simulink model "My_gfm_datacenter_sil"  (R2018b)
settings: Solver=ode45  StartTime=0.0  StopTime=100  MaxStep=1e-4  RelTol=1e-3
PreLoadFcn:
  | modelDir = fileparts(get_param(bdroot,'FileName'));
  | 
  | load_system(fullfile(modelDir,'controls_element_lib.slx'));
  | load_system(fullfile(modelDir,'test_sequence_lib.slx'));
InitFcn:
  | close all;
  | clear all;
  | clc;
  | 
  | % frequency nominals
  | F_NOM = 60;
  | W_NOM = 2 * pi * F_NOM;
  | 
  | % base values relative to inverter
  | % --------------------------------
  | VLL_INV_NOM = 480;
  | P_INV_NOM = 1e6;
  | Q_INV_NOM = 0.5e6;
  | S_INV_NOM = sqrt(P_INV_NOM^2 + Q_INV_NOM^2);
  | 
  | I_INV_BASE = S_INV_NOM/(sqrt(3)*VLL_INV_NOM);
  | Z_INV_BASE = VLL_INV_NOM^2/S_INV_NOM;
  | L_INV_BASE = Z_INV_BASE / W_NOM;
  | C_INV_BASE = 1 / (Z_INV_BASE * W_NOM);
  | 
  | % nominal ratings for power system model
  | % --------------------------------------
  | INVERTER_COUNT = 100;
  | 
  | VLV_NOM = VLL_INV_NOM;
  | VMV_NOM = 35e3;
  | VHV_NOM = 230e3;
  | S_PLANT = INVERTER_COUNT * S_INV_NOM;
  | 
  | N_GSU = VHV_NOM/VMV_NOM;
  | N_MVT = VMV_NOM/VLV_NOM;
  | 
  | I_LV_BASE = S_PLANT/(sqrt(3)*VLV_NOM);
  | I_MV_BASE = S_PLANT/(sqrt(3)*VMV_NOM);
  | I_HV_BASE = S_PLANT/(sqrt(3)*VHV_NOM);
  | 
  | Z_LV_BASE = VLV_NOM^2/S_PLANT;
  | Z_MV_BASE = VMV_NOM^2/S_PLANT;
  | Z_HV_BASE = VHV_NOM^2/S_PLANT;
  | 
  | L_LV_BASE = Z_LV_BASE / W_NOM;
  | L_MV_BASE = Z_MV_BASE / W_NOM;
  | L_HV_BASE = Z_HV_BASE / W_NOM;
  | C_LV_BASE = 1 / (Z_LV_BASE * W_NOM);
  | C_MV_BASE = 1 / (Z_MV_BASE * W_NOM);
  | C_HV_BASE = 1 / (Z_HV_BASE * W_NOM);
undefined symbols (not defined in the file): C_BBU, C_MV_CELL, IDC_NOM, ILV_MAX, ILV_MIN, IMV_MAX, IMV_MIN, N_CELLS_PER_STRING, N_DCDC_XFMR, r_BBU, V_LVDC_NOM
libraries: test_sequence_lib x14, controls_element_lib x10, simulink x1
settings Model: SimulationMode=accelerator  Creator=HussamAlatrash  LastModifiedBy=ahhei
settings DataIOCC: ReturnWorkspaceOutputs=on
settings OptimizationCC: EfficientMapNaN2IntZero=off
settings DebuggingCC: UnconnectedInputMsg=none  UnconnectedOutputMsg=none  UnconnectedLineMsg=none
settings HardwareCC: TargetBitPerPointer=64  TargetBitPerSizeT=64  TargetBitPerPtrDiffT=64  TargetLongLongMode=on  TargetIntDivRoundTo=Zero  TargetEndianess=LittleEndian  TargetWordSize=64  TargetHWDeviceType=MATLAB Host  ProdEqTarget=off
settings ModelReferenceCC: EnableRefExpFcnMdlSchedulingChecks=off
settings CodeAppCC: MaxIdLength=128
settings GRTTargetCC: TargetLangStandard=C89/C90 (ANSI)  CombineOutputUpdateFcns=off  GRTInterface=on

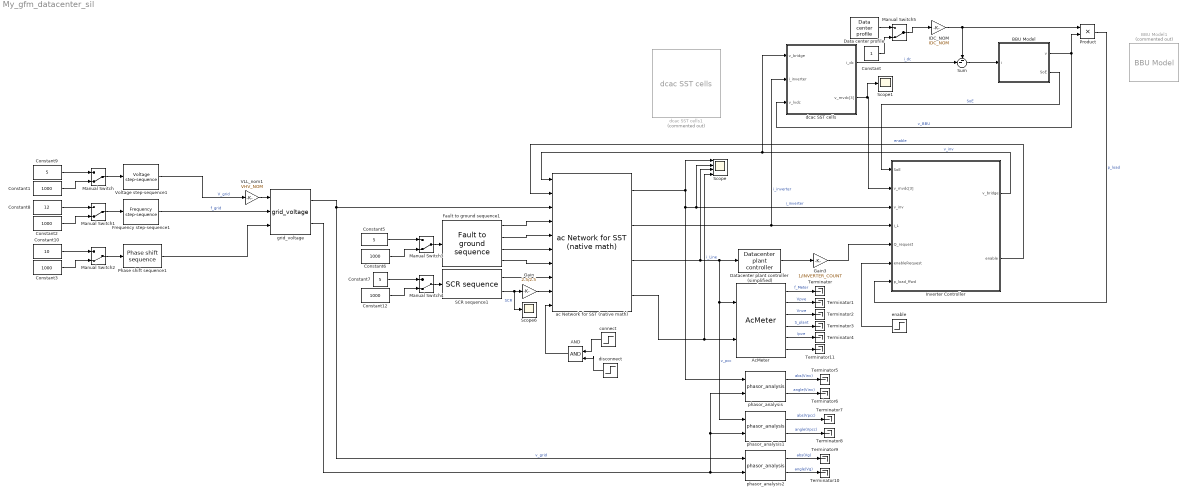
== system My_gfm_datacenter_sil ==
  AND : Logic  IconShape=distinctive  AllPortsSameDT=off  OutDataTypeStr=boolean
  AcMeter : test_sequence_lib/AcMeter  VllRated=VHV_NOM
  BBU Model : Subsystem  AncestorBlock=test_sequence_lib/BBU Model
  BBU Model1 : test_sequence_lib/BBU Model  Commented=on  SystemSampleTime=-1
  Constant : Constant
  Constant{1..3,6,12} (5 alike) : Constant  Value=1000
  Constant10 : Constant  Value=10
  Constant5 : Constant  Value=5
  Constant7 : Constant  Value=5
  Constant8 : Constant  Value=12
  Constant9 : Constant  Value=5
  Data center profile : test_sequence_lib/Data center profile  SystemSampleTime=-1
  Datacenter plant controller (simplified) : controls_element_lib/Datacenter plant controller  SystemSampleTime=-1
  Fault to ground sequence1 : test_sequence_lib/Fault to ground sequence  SystemSampleTime=-1
  Frequency step-sequence1 : test_sequence_lib/Frequency step-sequence  SystemSampleTime=-1
  Gain : Gain  Gain=2.5/2.5
  Gain3 : Gain  Gain=1/INVERTER_COUNT
  IDC_NOM : Gain  Gain=IDC_NOM
  Inverter Controller : Subsystem
  Manual Switch{,1..5} (6 alike) : ManualSwitch  CurrentSetting=0
  Phase shift sequence1 : test_sequence_lib/Phase shift sequence  SystemSampleTime=-1
  Product : Product
  SCR sequence1 : test_sequence_lib/SCR sequence  SystemSampleTime=-1
  Scope : Scope  NumInputPorts=4
  Scope1 : Scope
  Scope6 : Scope
  Sum : Sum  Inputs=--|
  Terminator{,1..11} (12 alike) : Terminator
  VLL_nom1 : Gain  Gain=VHV_NOM
  Voltage step-sequence1 : test_sequence_lib/Voltage step-sequence  SystemSampleTime=-1
  ac Network for SST (native math) : test_sequence_lib/ac Network for SST (native math)  SystemSampleTime=-1
  connect : Step  Time=0  SampleTime=0
  dcac SST cells : Subsystem  AncestorBlock=test_sequence_lib/dcac SST cells
  dcac SST cells1 : test_sequence_lib/dcac SST cells  Commented=on  SystemSampleTime=-1
  disconnect : Step  Time=97  Before=1  SampleTime=0
  enable : Step  Time=2  SampleTime=0
  grid_voltage : test_sequence_lib/grid_voltage  SystemSampleTime=-1
  phasor_analysis : test_sequence_lib/phasor_analysis  SystemSampleTime=-1
  phasor_analysis1 : test_sequence_lib/phasor_analysis  SystemSampleTime=-1
  phasor_analysis2 : test_sequence_lib/phasor_analysis  SystemSampleTime=-1
  wires:
  Data center profile/1 -> Manual Switch5/1
  Inverter Controller/2(enable) -> ac Network for SST (native math)/2  "enable"
  Constant9/1 -> Manual Switch/1
  Constant3/1 -> Manual Switch2/2
  VLL_nom1/1 -> grid_voltage/1
  Manual Switch3/1 -> Fault to ground sequence1/1
  Voltage step-sequence1/1 -> VLL_nom1/1  "V_grid"
  Constant/1 -> Manual Switch5/2
  Constant6/1 -> Manual Switch3/2
  Fault to ground sequence1/2 -> ac Network for SST (native math)/5
  ac Network for SST (native math)/4 -> Scope/4, AcMeter/2  "i_Line"
  ac Network for SST (native math)/1 -> Scope/2, Inverter Controller/3(v_inv), phasor_analysis/1, Scope/1  "i_inverter"
  Constant8/1 -> Manual Switch1/1
  Gain/1 -> ac Network for SST (native math)/9
  Inverter Controller/1(v_bridge) -> dcac SST cells/1(v_bridge), ac Network for SST (native math)/1  "v_inv"
  SCR sequence1/2 -> Scope6/1, Gain/1  "SCR"
  phasor_analysis1/2 -> Terminator8/1  "angle(Vpcc)"
  Constant1/1 -> Manual Switch/2
  Manual Switch5/1 -> IDC_NOM/1
  Fault to ground sequence1/1 -> ac Network for SST (native math)/4
  Frequency step-sequence1/1 -> grid_voltage/2  "f_grid"
  Constant5/1 -> Manual Switch3/1
  Fault to ground sequence1/4 -> ac Network for SST (native math)/7
  Fault to ground sequence1/3 -> ac Network for SST (native math)/6
  AcMeter/2 -> Terminator1/1  "Vpve"
  dcac SST cells/1(i_dc) -> Sum/2  "i_dc"
  phasor_analysis/1 -> Terminator5/1  "abs(Vinv)"
  AcMeter/4 -> Terminator3/1  "S_plant"
  Manual Switch/1 -> Voltage step-sequence1/1
  Manual Switch1/1 -> Frequency step-sequence1/1
  Datacenter plant controller (simplified)/1 -> Gain3/1
  connect/1 -> AND/1
  Phase shift sequence1/1 -> grid_voltage/3
  Constant10/1 -> Manual Switch2/1
  disconnect/1 -> AND/2
  ac Network for SST (native math)/2 -> Inverter Controller/4(i_L), dcac SST cells/2(i_inverter)  "i_inverter"
  dcac SST cells/2(v_mvdc[3]) -> Scope1/1, Inverter Controller/2(v_mvdc[3])
  AND/1 -> ac Network for SST (native math)/10
  enable/1 -> Inverter Controller/6(enableRequest)
  Constant7/1 -> Manual Switch4/1
  grid_voltage/2 -> phasor_analysis1/2, phasor_analysis/2, phasor_analysis2/2
  grid_voltage/1 -> ac Network for SST (native math)/3, phasor_analysis2/1  "v_grid"
  SCR sequence1/1 -> ac Network for SST (native math)/8
  phasor_analysis1/1 -> Terminator7/1  "abs(Vpcc)"
  ac Network for SST (native math)/3 -> Scope/3, Datacenter plant controller (simplified)/1, phasor_analysis1/1, AcMeter/1  "v_pcc"
  Constant12/1 -> Manual Switch4/2
  BBU Model/1(v) -> dcac SST cells/3(v_lvdc), Product/2  "v_BBU"
  IDC_NOM/1 -> Sum/1, Product/1
  phasor_analysis2/2 -> Terminator10/1  "angle(Vg)"
  Product/1 -> Inverter Controller/7(p_load_ffwd)  "p_load"
  BBU Model/2(SoE) -> Inverter Controller/1(SoE)  "SoE"
  Gain3/1 -> Inverter Controller/5(Q_request)
  phasor_analysis/2 -> Terminator6/1  "angle(Vinv)"
  AcMeter/3 -> Terminator2/1  "Vnve"
  AcMeter/5 -> Terminator4/1  "Ipve"
  Constant2/1 -> Manual Switch1/2
  phasor_analysis2/1 -> Terminator9/1  "abs(Vg)"
  Manual Switch4/1 -> SCR sequence1/1
  Sum/1 -> BBU Model/1(i)
  AcMeter/6 -> Terminator11/1
  AcMeter/1 -> Terminator/1  "f_Meter"
  Manual Switch2/1 -> Phase shift sequence1/1

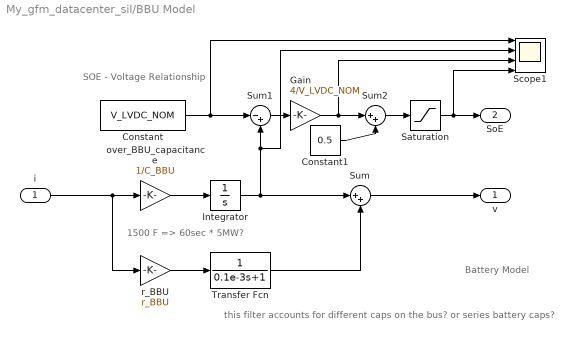
== system My_gfm_datacenter_sil/BBU Model ==
  note: Battery Model
  note: this filter accounts for different caps on the bus? or series battery caps?
  note: 1500 F => 60sec * 5MW?
  note: SOE - Voltage Relationship
  i : Inport
  Constant : Constant  Value=V_LVDC_NOM
  Constant1 : Constant  Value=0.5
  Gain : Gain  Gain=4/V_LVDC_NOM
  Integrator : Integrator  InitialCondition=V_LVDC_NOM
  Saturation : Saturate  UpperLimit=1.1  LowerLimit=-0.1
  Scope1 : Scope  NumInputPorts=4
  Sum : Sum  Inputs=|++
  Sum1 : Sum  Inputs=|-+
  Sum2 : Sum  Inputs=|++
  Transfer Fcn : TransferFcn  Denominator=[0.1e-3 1]
  over_BBU_capacitance : Gain  Gain=1/C_BBU
  r_BBU : Gain  Gain=r_BBU
  v : Outport  VectorParamsAs1DForOutWhenUnconnected=on
  SoE : Outport  Port=2  VectorParamsAs1DForOutWhenUnconnected=on
  wires:
  Saturation/1 -> Scope1/4, SoE/1
  Constant1/1 -> Sum2/2
  Sum2/1 -> Saturation/1
  Constant/1 -> Scope1/1, Sum1/1
  Sum1/1 -> Gain/1
  Gain/1 -> Scope1/3, Sum2/1
  Transfer Fcn/1 -> Sum/2
  Sum/1 -> v/1
  r_BBU/1 -> Transfer Fcn/1
  i/1 -> over_BBU_capacitance/1, r_BBU/1
  Integrator/1 -> Scope1/2, Sum1/2, Sum/1
  over_BBU_capacitance/1 -> Integrator/1

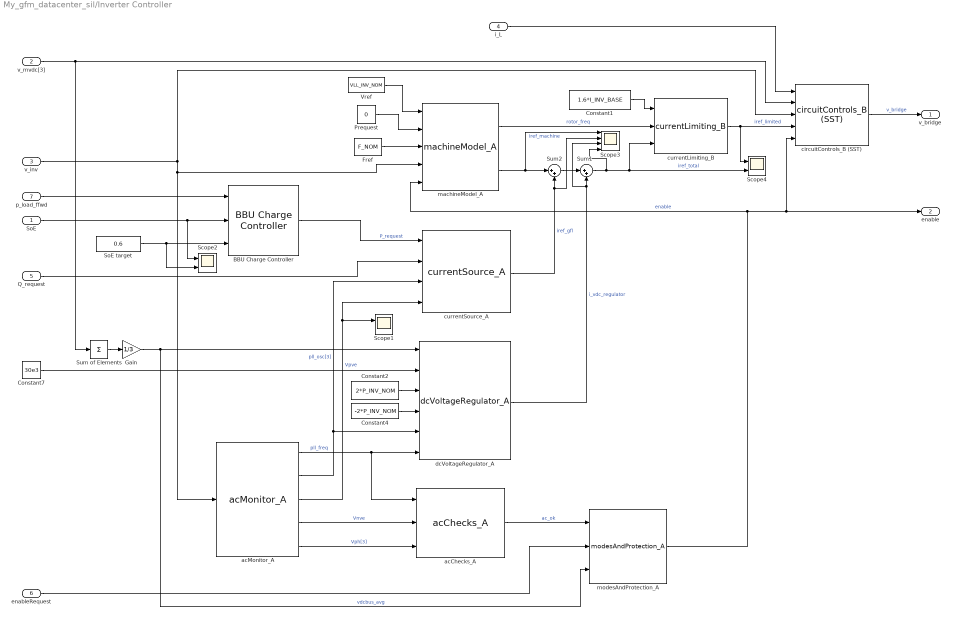
== system My_gfm_datacenter_sil/Inverter Controller ==
  SoE : Inport
  v_mvdc[3] : Inport  Port=2
  v_inv : Inport  Port=3
  i_L : Inport  Port=4
  Q_request : Inport  Port=5
  enableRequest : Inport  Port=6
  p_load_ffwd : Inport  Port=7
  BBU Charge Controller : controls_element_lib/BBU Charge Controller  SystemSampleTime=-1
  Constant1 : Constant  Value=1.6*I_INV_BASE
  Constant2 : Constant  Value=2*P_INV_NOM
  Constant4 : Constant  Value=-2*P_INV_NOM
  Constant7 : Constant  Value=30e3
  Fref : Constant  Value=F_NOM
  Gain : Gain  Gain=1/3
  Prequest : Constant  Value=0
  Scope1 : Scope  NumInputPorts=2
  Scope2 : Scope  NumInputPorts=2
  Scope3 : Scope  NumInputPorts=4
  Scope4 : Scope  NumInputPorts=2
  SoE target : Constant  Value=0.6
  Sum of Elements : Sum  Inputs=+
  Sum1 : Sum  Inputs=|++
  Sum2 : Sum  Inputs=|++
  Vref : Constant  Value=VLL_INV_NOM
  acChecks_A : controls_element_lib/acChecks_A  VllRated=VLL_INV_NOM  nominalFrequency=F_NOM  tRequalify=2  T_CNTL=1e-3
  acMonitor_A : controls_element_lib/acMonitor_A  VllRated=VLL_INV_NOM  nominalFrequency=F_NOM
  circuitControls_B (SST) : controls_element_lib/circuitControls_B (SST)  SystemSampleTime=-1
  currentLimiting_B : controls_element_lib/currentLimiting_B  IRated=I_INV_BASE  peakSoftLimit=2.6  peakHardLimit=3.6
  currentSource_A : controls_element_lib/currentSource_A  VllRated=VLL_INV_NOM  SRated=S_INV_NOM  nominalFrequency=F_NOM  Plimit=P_INV_NOM/S_INV_NOM  Qlimit=Q_INV_NOM/S_INV_NOM
  dcVoltageRegulator_A : controls_element_lib/dcVoltageRegulator_A  kp=5e3  kSlowPath=0  wSlowPath=5  pLimitExternalMinimum=0.05*P_INV_NOM  vdc_deadband=1500  VllRated=VLL_INV_NOM
  machineModel_A : controls_element_lib/machineModel_A  SRated=S_INV_NOM  VllRated=VLL_INV_NOM  nominalFrequency=F_NOM  inertialConstant=2.5  kDroop=1  kDamper=2  Xs=0.3  rs=0.08  Qlimit=0.5  wExciter=10
  modesAndProtection_A : controls_element_lib/modesAndProtection_A  dcOvervotlageThreshold=40e3  dcUndervotlageThreshold=23e3  dcTripClearTimeout=0.2
  v_bridge : Outport  VectorParamsAs1DForOutWhenUnconnected=on
  enable : Outport  Port=2  VectorParamsAs1DForOutWhenUnconnected=on
  wires:
  Vref/1 -> machineModel_A/1
  Prequest/1 -> machineModel_A/2
  Fref/1 -> machineModel_A/3
  machineModel_A/2 -> Scope3/1, Sum2/1  "iref_machine"
  currentLimiting_B/1 -> Scope4/1, circuitControls_B (SST)/4  "iref_limited"
  v_inv/1 -> circuitControls_B (SST)/3, acMonitor_A/1, machineModel_A/4
  currentSource_A/1 -> Scope3/2, Sum2/2  "iref_gfl"
  Sum1/1 -> Scope3/4, Scope4/2, currentLimiting_B/3  "iref_total"
  acMonitor_A/2 -> currentSource_A/3, dcVoltageRegulator_A/5  "pll_osc[3]"
  Q_request/1 -> currentSource_A/2
  acMonitor_A/4 -> acChecks_A/2  "Vnve"
  enableRequest/1 -> modesAndProtection_A/2
  modesAndProtection_A/1 -> machineModel_A/5, enable/1, circuitControls_B (SST)/5  "enable"
  BBU Charge Controller/1 -> currentSource_A/1  "P_request"
  acMonitor_A/3 -> Scope1/1, currentSource_A/4  "Vpve"
  Constant1/1 -> currentLimiting_B/1
  acMonitor_A/5 -> acChecks_A/3  "Vph[3]"
  acChecks_A/1 -> modesAndProtection_A/1  "ac_ok"
  acMonitor_A/1 -> dcVoltageRegulator_A/6, acChecks_A/1  "pll_freq"
  dcVoltageRegulator_A/1 -> Scope3/3, Sum1/2  "i_vdc_regulator"
  Sum2/1 -> Sum1/1
  Constant7/1 -> dcVoltageRegulator_A/2
  Sum of Elements/1 -> Gain/1
  Gain/1 -> modesAndProtection_A/3, dcVoltageRegulator_A/1  "vdcbus_avg"
  Constant2/1 -> dcVoltageRegulator_A/3
  Constant4/1 -> dcVoltageRegulator_A/4
  SoE/1 -> Scope2/1, BBU Charge Controller/2
  p_load_ffwd/1 -> BBU Charge Controller/1
  circuitControls_B (SST)/1 -> v_bridge/1  "v_bridge"
  v_mvdc[3]/1 -> Sum of Elements/1, circuitControls_B (SST)/2
  i_L/1 -> circuitControls_B (SST)/1
  SoE target/1 -> Scope2/2, BBU Charge Controller/3
  machineModel_A/1 -> currentLimiting_B/2  "rotor_freq"

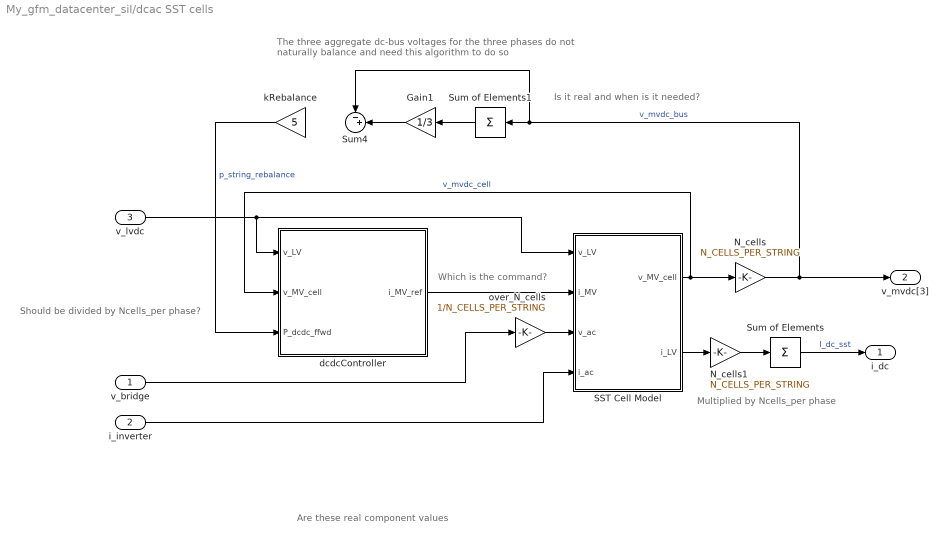
== system My_gfm_datacenter_sil/dcac SST cells ==
  note: Should be divided by Ncells_per phase?
  note: The three aggregate dc-bus voltages for the three phases do not naturally balance and need this algorithm to do so
  note: Multiplied by Ncells_per phase
  note: Which is the command?
  note: Is it real and when is it needed?
  note: Are these real component values
  v_bridge : Inport
  i_inverter : Inport  Port=2
  v_lvdc : Inport  Port=3
  Gain1 : Gain  Gain=1/3
  N_cells : Gain  Gain=N_CELLS_PER_STRING
  N_cells1 : Gain  Gain=N_CELLS_PER_STRING
  SST Cell Model : Subsystem
  Sum of Elements : Sum  Inputs=+
  Sum of Elements1 : Sum  Inputs=+
  Sum4 : Sum  Inputs=-+|
  dcdcController : Subsystem
  kRebalance : Gain  Gain=5
  over_N_cells : Gain  Gain=1/N_CELLS_PER_STRING
  i_dc : Outport  VectorParamsAs1DForOutWhenUnconnected=on
  v_mvdc[3] : Outport  Port=2  VectorParamsAs1DForOutWhenUnconnected=on
  wires:
  i_inverter/1 -> SST Cell Model/4(i_ac)
  Sum of Elements/1 -> i_dc/1  "I_dc_sst"
  v_bridge/1 -> over_N_cells/1
  v_lvdc/1 -> dcdcController/1(v_LV), SST Cell Model/1(v_LV)
  over_N_cells/1 -> SST Cell Model/3(v_ac)
  SST Cell Model/1(v_MV_cell) -> dcdcController/2(v_MV_cell), N_cells/1  "v_mvdc_cell"
  Gain1/1 -> Sum4/2
  dcdcController/1(i_MV_ref) -> SST Cell Model/2(i_MV)
  Sum of Elements1/1 -> Gain1/1
  SST Cell Model/2(i_LV) -> N_cells1/1
  N_cells/1 -> Sum of Elements1/1, Sum4/1, v_mvdc[3]/1  "v_mvdc_bus"
  N_cells1/1 -> Sum of Elements/1
  kRebalance/1 -> dcdcController/3(P_dcdc_ffwd)  "p_string_rebalance"

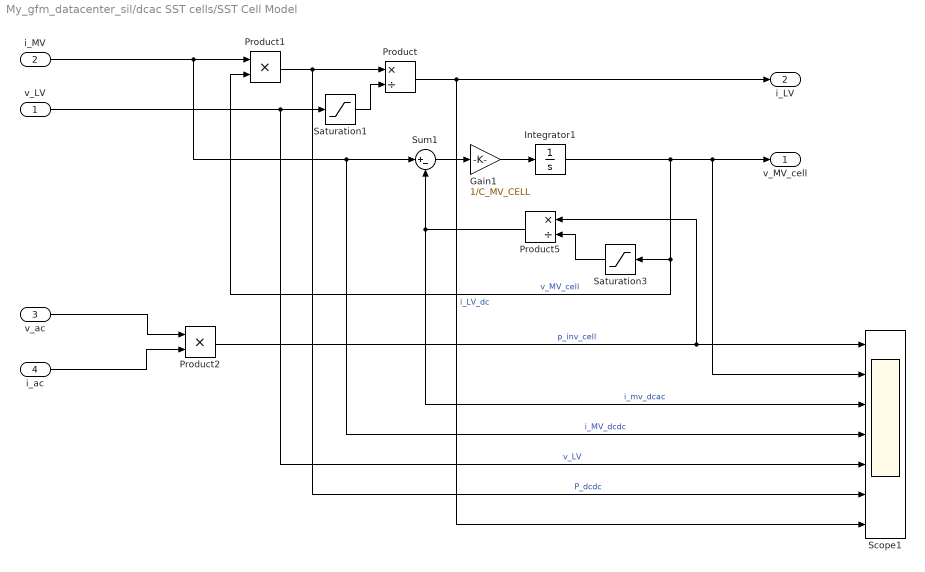
== system My_gfm_datacenter_sil/dcac SST cells/SST Cell Model ==
  v_LV : Inport
  i_MV : Inport  Port=2
  v_ac : Inport  Port=3
  i_ac : Inport  Port=4
  Gain1 : Gain  Gain=1/C_MV_CELL
  Integrator1 : Integrator
  Product : Product  Inputs=*/
  Product1 : Product
  Product2 : Product
  Product5 : Product  Inputs=*/
  Saturation1 : Saturate  UpperLimit=inf  LowerLimit=50
  Saturation3 : Saturate  UpperLimit=inf  LowerLimit=500
  Scope1 : Scope  NumInputPorts=7
  Sum1 : Sum  Inputs=|+-
  v_MV_cell : Outport  VectorParamsAs1DForOutWhenUnconnected=on
  i_LV : Outport  Port=2  VectorParamsAs1DForOutWhenUnconnected=on
  wires:
  Saturation1/1 -> Product/2
  Product/1 -> Scope1/7, i_LV/1  "i_LV_dc"
  v_ac/1 -> Product2/1
  i_ac/1 -> Product2/2
  Product2/1 -> Product5/1, Scope1/1  "p_inv_cell"
  i_MV/1 -> Scope1/4, Sum1/1, Product1/1  "i_MV_dcdc"
  Sum1/1 -> Gain1/1
  Product1/1 -> Scope1/6, Product/1  "P_dcdc"
  Product5/1 -> Scope1/3, Sum1/2  "i_mv_dcac"
  Gain1/1 -> Integrator1/1
  v_LV/1 -> Scope1/5, Saturation1/1  "v_LV"
  Saturation3/1 -> Product5/2
  Integrator1/1 -> Product1/2, Saturation3/1, Scope1/2, v_MV_cell/1  "v_MV_cell"

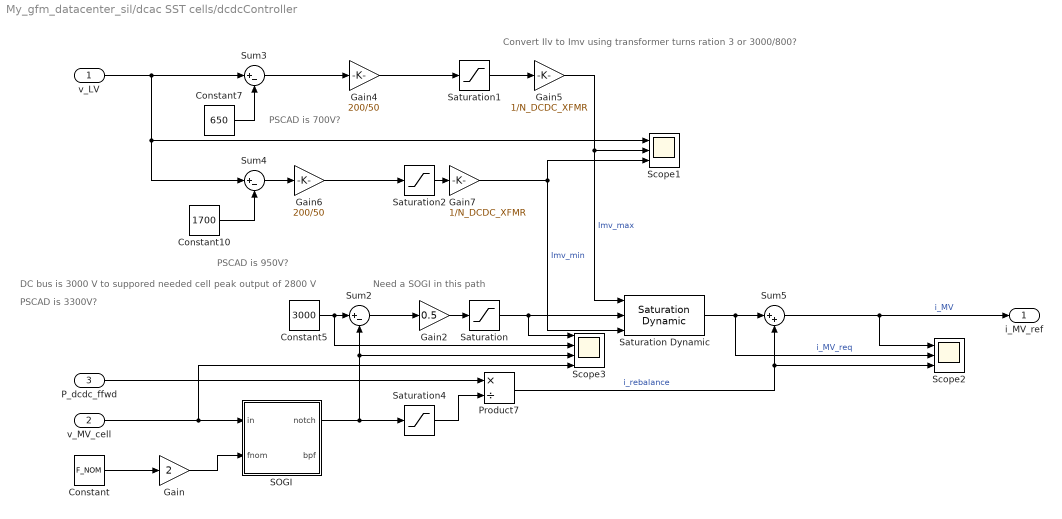
== system My_gfm_datacenter_sil/dcac SST cells/dcdcController ==
  note: Convert Ilv to Imv using transformer turns ration 3 or 3000/800?
  note: DC bus is 3000 V to suppored needed cell peak output of 2800 V
  note: Need a SOGI in this path
  note: PSCAD is 3300V?
  note: PSCAD is 700V?
  note: PSCAD is 950V?
  v_LV : Inport
  v_MV_cell : Inport  Port=2
  P_dcdc_ffwd : Inport  Port=3
  Constant : Constant  Value=F_NOM
  Constant10 : Constant  Value=1700
  Constant5 : Constant  Value=3000
  Constant7 : Constant  Value=650
  Gain : Gain  Gain=2
  Gain2 : Gain  Gain=0.5
  Gain4 : Gain  Gain=200/50
  Gain5 : Gain  Gain=1/N_DCDC_XFMR
  Gain6 : Gain  Gain=200/50
  Gain7 : Gain  Gain=1/N_DCDC_XFMR
  Product7 : Product  Inputs=*/
  SOGI : Subsystem
  Saturation : Saturate  UpperLimit=IMV_MAX  LowerLimit=IMV_MIN
  Saturation Dynamic : simulink/Discontinuities/Saturation Dynamic  OutMin=[]  OutMax=[]  OutDataTypeStr=Inherit: Same as second input  OutDataType=fixdt(1, 16)  OutScaling=2^-10  DoSatur=off
  Saturation1 : Saturate  UpperLimit=ILV_MAX  LowerLimit=ILV_MIN
  Saturation2 : Saturate  UpperLimit=ILV_MAX  LowerLimit=ILV_MIN
  Saturation4 : Saturate  UpperLimit=inf  LowerLimit=2000
  Scope1 : Scope  NumInputPorts=3
  Scope2 : Scope  NumInputPorts=3
  Scope3 : Scope  NumInputPorts=4
  Sum2 : Sum  Inputs=|+-
  Sum3 : Sum  Inputs=|+-
  Sum4 : Sum  Inputs=|+-
  Sum5 : Sum  Inputs=|++
  i_MV_ref : Outport  VectorParamsAs1DForOutWhenUnconnected=on
  wires:
  Constant/1 -> Gain/1
  v_MV_cell/1 -> Scope3/4, SOGI/1(in)
  Gain/1 -> SOGI/2(fnom)
  Sum5/1 -> Scope2/1, i_MV_ref/1  "i_MV"
  Saturation4/1 -> Product7/2
  Sum3/1 -> Gain4/1
  Saturation2/1 -> Gain7/1
  Gain5/1 -> Saturation Dynamic/1, Scope1/2  "Imv_max"
  P_dcdc_ffwd/1 -> Product7/1
  Gain7/1 -> Saturation Dynamic/3, Scope1/3  "Imv_min"
  Product7/1 -> Scope2/3, Sum5/2  "i_rebalance"
  Gain6/1 -> Saturation2/1
  Sum4/1 -> Gain6/1
  Saturation Dynamic/1 -> Scope2/2, Sum5/1  "i_MV_req"
  Saturation1/1 -> Gain5/1
  Constant5/1 -> Scope3/2, Sum2/1
  v_LV/1 -> Scope1/1, Sum4/1, Sum3/1
  Constant7/1 -> Sum3/2
  Gain2/1 -> Saturation/1
  Saturation/1 -> Scope3/1, Saturation Dynamic/2
  Gain4/1 -> Saturation1/1
  SOGI/1(notch) -> Saturation4/1, Sum2/2, Scope3/3
  Sum2/1 -> Gain2/1
  Constant10/1 -> Sum4/2

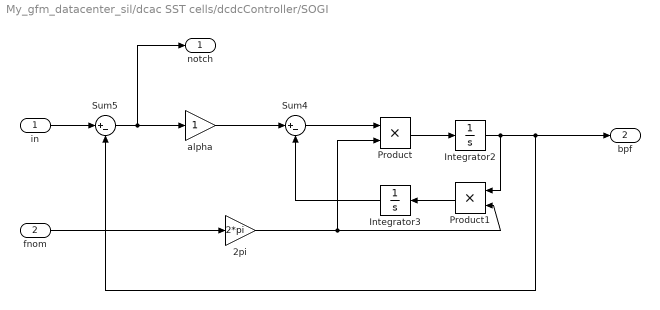
== system My_gfm_datacenter_sil/dcac SST cells/dcdcController/SOGI ==
  in : Inport
  fnom : Inport  Port=2
  2pi : Gain  Gain=2*pi
  Integrator2 : Integrator
  Integrator3 : Integrator
  Product : Product
  Product1 : Product
  Sum4 : Sum  Inputs=|+-
  Sum5 : Sum  Inputs=|+-
  alpha : Gain
  notch : Outport  VectorParamsAs1DForOutWhenUnconnected=on
  bpf : Outport  Port=2  VectorParamsAs1DForOutWhenUnconnected=on
  wires:
  in/1 -> Sum5/1
  fnom/1 -> 2pi/1
  Integrator2/1 -> Product1/1, Sum5/2, bpf/1
  alpha/1 -> Sum4/1
  Sum5/1 -> alpha/1, notch/1
  Sum4/1 -> Product/1
  Integrator3/1 -> Sum4/2
  2pi/1 -> Product1/2, Product/2
  Product/1 -> Integrator2/1
  Product1/1 -> Integrator3/1
